simulink library "ConverterPlantLibrary"  (R2026a)
settings: Solver=VariableStepAuto
libraries: nesl_utility x213, fl_lib x211, ee_lib x205
(part 16 of 22)

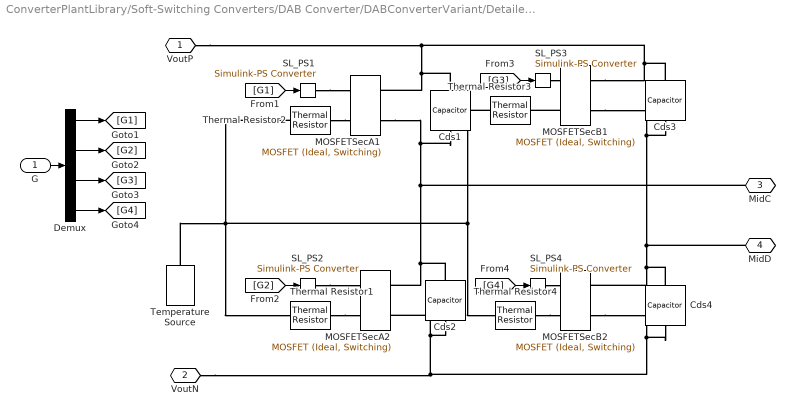
== system ConverterPlantLibrary/Soft-Switching Converters/DAB Converter/DABConverterVariant/DetailedModel/SecondaryBridge/SwitchingMOSFETwithThermal ==
  G : Inport
  Cds{1..4} (4 alike) : ee_lib/Passive/Capacitor  cap_option=ee.enum.passive.capacitor.capOption.const  c=CossSec_SI F  Cvec=[1e-05, 1e-06] F  Vvec=[0, 10] V  CV_table_symmetry=ee.enum.passive.capacitor.tableSymmetry.yes  f_vec=[1, 10] kHz  DFext_vec=[.8, 1.2]  enable_C_tol=ee.enum.toleranceApplication.none  averaging_period=0 s  C_tol=5  tol_distribution=ee.enum.toleranceDistribution.uniform  nSigma=4  r=0.001 Ohm  g=1e-5 1/Ohm  enable_operating_limits=ee.enum.enable.no  operating_limit_action=ee.enum.passive.reportOpLim.warn  max_working_voltage_range=[-25, 25] V  power_rating=1 W  maxTemperature=85 degC  thermalEnable=false  thermalMass=1 J/K  i_specify=off  i_priority=None  i=0 A  i_nominal_specify=off  i_nominal_value=1  i_nominal_unit=A  v_specify=off  v_priority=None  v=0 V  v_nominal_specify=off  v_nominal_value=1  v_nominal_unit=V  vc_specify=on  vc_priority=None  vc=0 V  vc_nominal_specify=off  vc_nominal_value=1  vc_nominal_unit=V  T_specify=off  T_priority=None  T=298.15 K  T_nominal_specify=off  T_nominal_value=1  T_nominal_unit=K
  Demux : Demux
  MOSFETSecA1 : ee_lib/Semiconductors & Converters/MOSFET (Ideal, Switching)  PartSpecification="{\"CollectionId\":\"MW.SimscapeElectrical\",\"CollectionVersion\":\"1.0.0\",\"DatasetId\":\"Wolfspeed|E4M0045075K1|\",\"DisplayName\":\"Wolfspeed:E4M0045075K1\"}"  port_option=ee.enum.controlport.ps  Rds=0.045 % Datasheet derived Ohm  Goff=1e-05 S  Vth=2.6 % Wolfspeed XML derived V  diode_param=ee.enum.converters.protectiondiode.nodynamics  diode_Vf=2.21 % Datasheet derived V  diode_Ron=0.02 % Wolfspeed XML derived Ohm  diode_Goff=1e-05 % Library default S  diode_C=50e-9 % Parameter not set F  diode_iRM=-235 % Parameter not set A  diode_iF=300 % Parameter not set A  diode_idot=-50 % Parameter not set A/us  diode_trr_param=ee.enum.converters.diodeReverseParam.trr_factor  diode_trr_factor=3 % Parameter not set  diode_trr=15 % Parameter not set us  diode_Qrr=1500 % Parameter not set s*uA  ids_specify=off  ids_priority=None  ids=0 A  ids_nominal_specify=off  ids_nominal_value=1  ids_nominal_unit=A  vds_specify=off  vds_priority=None  vds=0 V  vds_nominal_specify=off  vds_nominal_value=1  vds_nominal_unit=V  vgs_specify=off  vgs_priority=None  vgs=0 V  vgs_nominal_specify=off  vgs_nominal_value=1  vgs_nominal_unit=V  thermal_loss_option=ee.enum.converters.thermalLossOption.tabulated2d  Von_data=[-4.5606 -3.8186 -3.2298 -2.6407 -2.0162 -1.3202 -0.71619 -0.4914 -0.25251 -0.10121 -0.049071 0 0.046955 0.096318 0.24814 0.51166 0.78533 1.638 2.8067 4.0083;-6.1438 -4.6059 -3.5721 -2.779 -2.0216 -1.2551 -0.64969 -0.43829 -0.22166 -0.088463 -0.0434 0 0.04287 0.088364 0.22316 0.45399 0.69097 1.4423 2.5474 3.8258;-8.4687 -7.7777 -6.5652 -4.9559 -3.3669 -1.9919 -1.0021 -0.67224 -0.33819 -0.13631 -0.067471 0 0.066975 0.13508 0.34144 0.68685 1.0406 2.1699 3.9874 6.6428;-9.3156 -8.5555 -7.2218 -5.4514 -3.7036 -2.1911 -1.1023 -0.73946 -0.37201 -0.14994 -0.074218 0 0.073673 0.14859 0.37559 0.75553 1.1447 2.3869 4.3861 7.3071] % Wolfspeed XML derived V  Tj=[-55 25 175 900] % Wolfspeed XML derived degC  Iout_data=[-130 -110 -90 -70 -50 -30 -15 -10 -5 -2 -1 0 1 2 5 10 15 30 50 70] % Wolfspeed XML derived A  tabulateWithVds=false  Eon_data=[0 7.0888e-05 7.7152e-05 8.1716e-05 8.4697e-05 8.7728e-05 9.0888e-05 9.4243e-05 9.744e-05;0 7.7446e-05 8.2187e-05 8.4859e-05 8.6481e-05 8.8862e-05 9.0056e-05 9.2324e-05 9.4668e-05;0 7.794e-05 8.1085e-05 8.3317e-05 8.3898e-05 8.5847e-05 8.7874e-05 9.064e-05 9.3256e-05;0 7.7083e-05 7.9013e-05 8.0167e-05 8.1936e-05 8.4209e-05 8.8203e-05 9.1018e-05 9.9494e-05;0 8.4792e-05 8.6915e-05 8.8184e-05 9.013e-05 9.263e-05 9.7023e-05 0.00010012 0.00010944] % Wolfspeed XML derived J  Eoff_data=[0 2.4146e-05 1.5297e-05 1.3888e-05 1.7201e-05 2.1289e-05 2.6159e-05 3.3682e-05 4.1813e-05;0 2.543e-05 1.8251e-05 1.4144e-05 1.9418e-05 2.3393e-05 2.9608e-05 3.7025e-05 4.5856e-05;0 2.3401e-05 1.8149e-05 1.3882e-05 1.8943e-05 2.3112e-05 2.887e-05 3.79e-05 4.7249e-05;0 2.4371e-05 1.7115e-05 1.4404e-05 1.9523e-05 2.3993e-05 3.0691e-05 3.9068e-05 4.987e-05;0 2.6808e-05 1.8827e-05 1.5845e-05 2.1475e-05 2.6393e-05 3.376e-05 4.2974e-05 5.4857e-05] % Wolfspeed XML derived J  Eon_data_3D=reshape([0;0;0;0;0;0;0;0;0;0;0;0;0;0;0;0;0;0;0;0;0;0;0;0;0;0;0;0;0;0;0;0;0;0;0;0;0;0;0;0;0;0;0;0;0;0;0;0;0;0;0;0;0;0;0;0;0;0;0;0;0;0;0;0;0;0;0;0;0;0;0;0;0;0;0;0;0;0;0;0;0;0;0;0;0;0;0;0;0;0;0;0;0;0;0;7.0888e-05;7.7446e-05;7.794e-05;7.7083e-05;8.4792e-05;7.7152e-05;8.2187e-05;8.1085e-05;7.9013e-05;8.6915e-05;8.1716e-05;8.4859e-05;8.3317e-05;8.0167e-05;8.8184e-05;8.4697e-05;8.6481e-05;8.3898e-05;8.1936e-05;9.013e-05;8.7728e-05;8.8862e-05;8.5847e-05;8.4209e-05;9.263e-05;9.0888e-05;9.0056e-05;8.7874e-05;8.8203e-05;9.7023e-05;9.4243e-05;9.2324e-05;9.064e-05;9.1018e-05;0.00010012;9.744e-05;9.4668e-05;9.3256e-05;9.9494e-05;0.00010944],[5 9 3]) % Wolfspeed XML derived J  Eoff_data_3D=reshape([0;0;0;0;0;0;0;0;0;0;0;0;0;0;0;0;0;0;0;0;0;0;0;0;0;0;0;0;0;0;0;0;0;0;0;0;0;0;0;0;0;0;0;0;0;0;0;0;0;0;0;0;0;0;0;0;0;0;0;0;0;0;0;0;0;0;0;0;0;0;0;0;0;0;0;0;0;0;0;0;0;0;0;0;0;0;0;0;0;0;0;0;0;0;0;2.4146e-05;2.543e-05;2.3401e-05;2.4371e-05;2.6808e-05;1.5297e-05;1.8251e-05;1.8149e-05;1.7115e-05;1.8827e-05;1.3888e-05;1.4144e-05;1.3882e-05;1.4404e-05;1.5845e-05;1.7201e-05;1.9418e-05;1.8943e-05;1.9523e-05;2.1475e-05;2.1289e-05;2.3393e-05;2.3112e-05;2.3993e-05;2.6393e-05;2.6159e-05;2.9608e-05;2.887e-05;3.0691e-05;3.376e-05;3.3682e-05;3.7025e-05;3.79e-05;3.9068e-05;4.2974e-05;4.1813e-05;4.5856e-05;4.7249e-05;4.987e-05;5.4857e-05],[5 9 3]) % Wolfspeed XML derived J  Tj_loss=[25 75 125 175 900] % Wolfspeed XML derived degC  Iout_data_loss=[0 4.78844 9.555 13.3613 17.6794 21.5425 25.5456 29.2381 32.9963] % Wolfspeed XML derived A  Vds_loss=[-100 0 500] % Wolfspeed XML derived V  Eon_scalar=22.86e-3 % Parameter not set J  Eoff_scalar=17.14e-3 % Parameter not set J  Voff=300 % Parameter not set V  Iout_scalar=600 % Parameter not set A  useCurrentFromPreviousCycle=false % Parameter not set  useVoltageFromPreviousCycle=false % Parameter not set  diodeModelType=ee.enum.converters.diodeModelType.tabulated  diodeTableType=ee.enum.diode.tableType.VfMat  diode_ReverseIVType=ee.enum.diode.diodeReverseIV.constant  diode_IfMat=[.07, .12, .19, 1.75, 4.24, 7.32, 11.2; .16, .3, .72, 2.14, 4.02, 6.35, 9.12] % Parameter not set A  diode_VfMat=[0 3.93919 4.34166 5.03764 5.72176 6.19029 7.12243 7.9435 8.58508 9.13853 9.62104 10.0233;0 3.40354 3.71573 4.29235 4.91641 5.38167 6.38957 7.34226 8.07348 8.65657 9.13334 9.54153;0 2.99679 3.29251 3.84591 4.43945 4.88555 5.86847 6.80976 7.53945 8.14153 8.65715 9.11245;0 2.39743 2.63401 3.07672 3.55156 3.90844 4.69478 5.44781 6.03156 6.51323 6.92572 7.28996] % Wolfspeed XML derived V  diode_TjVec=[-55 25 175 900] % Wolfspeed XML derived degC  diode_VfVec=[.5, .7, .9, 1.3, 1.7, 2.1, 2.5] % Parameter not set V  diode_IfVec=[0 1 2 5 10 15 30 50 70 90 110 130] % Wolfspeed XML derived A  diode_IrMat=[1e-06, 2e-06, 5e-06, 1e-05, 2.5e-05, 5e-05, .0001; 2e-06, 5e-06, 1e-05, 4e-05, 8e-05, .0002, .0005] % Parameter not set A  diode_VrMat=[10, 100, 200, 250, 300, 325, 350; 10, 70, 160, 220, 270, 300, 320] % Parameter not set V  diode_VrVec=[10, 20, 40, 50, 70, 80, 100] % Parameter not set V  diode_IrVec=[1e-06, 2e-06, 5e-06, 1e-05, 2e-05, 5e-05, .0001] % Parameter not set A  diode_Vr=-600 % Parameter not set V  diode_Ls=150 % Parameter not set nH  diode_Erec=0.03 % Parameter not set J  diode_rec_loss_model=ee.enum.diode.reverseRecoveryModel.fixed  diode_ErecVal=0 % Parameter not set J  diode_scaleWithIandV=false  diode_ErecMat=[0 0;0 0] % Wolfspeed XML derived J  diodeErecMat3D=zeros(2, 3, 2) J  diode_TjrecVec=[25 35] % Wolfspeed XML derived degC  diode_IfrecVec=[0 10] % Wolfspeed XML derived A  diodeVrecVec=[0, 100] V  diode_IrecVal=10 % Parameter not set A  diode_VrecVal=10 % Wolfspeed XML derived V  diode_tFilter=1 / 1000 / 100 % Parameter not set s  separateThermalPortForDiode=false  thermal_network_parameterization=ee.enum.thermalNetworkTopology.external  Rth=[.03, .2] % Parameter not set K/W  Rth_Cauer=[0.089671 0.30799 0.22252 0.20902] % Wolfspeed XML derived K/W  Rth_Foster=[.08, .14, .22, .16] % Parameter not set K/W  thermal_mass_parameterization=ee.enum.thermalNetwork.thermalmass  thermal_mass=[3, 25] % Parameter not set J/K  thermal_mass_Cauer=[0.00092793 0.0041354 0.020593 0.15749] % Wolfspeed XML derived J/K  thermal_mass_Foster=[.001, .005, .05, .5] % Parameter not set J/K  thermal_time_constant=[.1, 5] % Parameter not set s  thermal_time_constant_Cauer=[.1, 1, 5] % Parameter not set s  thermal_time_constant_Foster=[7e-05, .0007, .01, .08] % Parameter not set s  thermal_mass_initial_temperatures=[25, 25] % Parameter not set degC  thermal_mass_initial_temperatures_Cauer=[25 25 25 25] % Wolfspeed XML derived degC  junction_thermal_mass=0.1 % Parameter not set J/K  Tvec_initial_Foster=[25, 25, 25, 25] % Parameter not set degC  RthDiode=[.03, .2] % Parameter not set K/W  RthCauerDiode=[0.089671 0.30799 0.22252 0.20902] % Wolfspeed XML derived K/W  RthFosterDiode=[.03, .2] % Parameter not set K/W  thermalMassDiode=[3, 25] % Parameter not set J/K  thermalMassCauerDiode=[0.00092793 0.0041354 0.020593 0.15749] % Wolfspeed XML derived J/K  thermalMassFosterDiode=[33, 50] % Parameter not set J/K  thermalTauDiode=[.1, 5] % Parameter not set s  thermalTauCauerDiode=[.1, 1, 5] % Parameter not set s  thermalTauFosterDiode=[1, 10] % Parameter not set s  thermalMassInitTempDiode=[25, 25] % Parameter not set degC  thermalMassInitTempCauerDiode=[25 25 25 25] % Wolfspeed XML derived degC  junctionthermalMassDiode=0.1 % Parameter not set J/K  TVecInitialFosterDiode=[25, 25, 25, 25] % Parameter not set degC  no_thermal_network=0 % Parameter not set  mosfet_junction_temperature_specify=on  mosfet_junction_temperature_priority=High  mosfet_junction_temperature=simTempSec_K K  mosfet_junction_temperature_nominal_specify=off  mosfet_junction_temperature_nominal_value=1  mosfet_junction_temperature_nominal_unit=degC  diode_junction_temperature_specify=off  diode_junction_temperature_priority=None  diode_junction_temperature=simTempSec_K K  diode_junction_temperature_nominal_specify=off  diode_junction_temperature_nominal_value=1  diode_junction_temperature_nominal_unit=degC  Qj_specify=off  Qj_priority=None  Qj=0 W  Qj_nominal_specify=off  Qj_nominal_value=1  Qj_nominal_unit=W  accumulatedSwitchingLosses_specify=off  accumulatedSwitchingLosses_priority=None  accumulatedSwitchingLosses=0 J
      settings: AttributesFormatString=Wolfspeed:E4M0045075K1
  MOSFETSecA2 : ee_lib/Semiconductors & Converters/MOSFET (Ideal, Switching)  port_option=ee.enum.controlport.ps  Rds=0.045 % Datasheet derived Ohm  Goff=1e-05 S  Vth=2.6 % Wolfspeed XML derived V  diode_param=ee.enum.converters.protectiondiode.nodynamics  diode_Vf=2.21 % Datasheet derived V  diode_Ron=0.02 % Wolfspeed XML derived Ohm  diode_Goff=1e-05 % Library default S  diode_C=50e-9 % Parameter not set F  diode_iRM=-235 % Parameter not set A  diode_iF=300 % Parameter not set A  diode_idot=-50 % Parameter not set A/us  diode_trr_param=ee.enum.converters.diodeReverseParam.trr_factor  diode_trr_factor=3 % Parameter not set  diode_trr=15 % Parameter not set us  diode_Qrr=1500 % Parameter not set s*uA  ids_specify=off  ids_priority=None  ids=0 A  ids_nominal_specify=off  ids_nominal_value=1  ids_nominal_unit=A  vds_specify=off  vds_priority=None  vds=0 V  vds_nominal_specify=off  vds_nominal_value=1  vds_nominal_unit=V  vgs_specify=off  vgs_priority=None  vgs=0 V  vgs_nominal_specify=off  vgs_nominal_value=1  vgs_nominal_unit=V  thermal_loss_option=ee.enum.converters.thermalLossOption.tabulated2d  Von_data=[-4.5606 -3.8186 -3.2298 -2.6407 -2.0162 -1.3202 -0.71619 -0.4914 -0.25251 -0.10121 -0.049071 0 0.046955 0.096318 0.24814 0.51166 0.78533 1.638 2.8067 4.0083;-6.1438 -4.6059 -3.5721 -2.779 -2.0216 -1.2551 -0.64969 -0.43829 -0.22166 -0.088463 -0.0434 0 0.04287 0.088364 0.22316 0.45399 0.69097 1.4423 2.5474 3.8258;-8.4687 -7.7777 -6.5652 -4.9559 -3.3669 -1.9919 -1.0021 -0.67224 -0.33819 -0.13631 -0.067471 0 0.066975 0.13508 0.34144 0.68685 1.0406 2.1699 3.9874 6.6428;-9.3156 -8.5555 -7.2218 -5.4514 -3.7036 -2.1911 -1.1023 -0.73946 -0.37201 -0.14994 -0.074218 0 0.073673 0.14859 0.37559 0.75553 1.1447 2.3869 4.3861 7.3071] % Wolfspeed XML derived V  Tj=[-55 25 175 900] % Wolfspeed XML derived degC  Iout_data=[-130 -110 -90 -70 -50 -30 -15 -10 -5 -2 -1 0 1 2 5 10 15 30 50 70] % Wolfspeed XML derived A  tabulateWithVds=false  Eon_data=[0 7.0888e-05 7.7152e-05 8.1716e-05 8.4697e-05 8.7728e-05 9.0888e-05 9.4243e-05 9.744e-05;0 7.7446e-05 8.2187e-05 8.4859e-05 8.6481e-05 8.8862e-05 9.0056e-05 9.2324e-05 9.4668e-05;0 7.794e-05 8.1085e-05 8.3317e-05 8.3898e-05 8.5847e-05 8.7874e-05 9.064e-05 9.3256e-05;0 7.7083e-05 7.9013e-05 8.0167e-05 8.1936e-05 8.4209e-05 8.8203e-05 9.1018e-05 9.9494e-05;0 8.4792e-05 8.6915e-05 8.8184e-05 9.013e-05 9.263e-05 9.7023e-05 0.00010012 0.00010944] % Wolfspeed XML derived J  Eoff_data=[0 2.4146e-05 1.5297e-05 1.3888e-05 1.7201e-05 2.1289e-05 2.6159e-05 3.3682e-05 4.1813e-05;0 2.543e-05 1.8251e-05 1.4144e-05 1.9418e-05 2.3393e-05 2.9608e-05 3.7025e-05 4.5856e-05;0 2.3401e-05 1.8149e-05 1.3882e-05 1.8943e-05 2.3112e-05 2.887e-05 3.79e-05 4.7249e-05;0 2.4371e-05 1.7115e-05 1.4404e-05 1.9523e-05 2.3993e-05 3.0691e-05 3.9068e-05 4.987e-05;0 2.6808e-05 1.8827e-05 1.5845e-05 2.1475e-05 2.6393e-05 3.376e-05 4.2974e-05 5.4857e-05] % Wolfspeed XML derived J  Eon_data_3D=reshape([0;0;0;0;0;0;0;0;0;0;0;0;0;0;0;0;0;0;0;0;0;0;0;0;0;0;0;0;0;0;0;0;0;0;0;0;0;0;0;0;0;0;0;0;0;0;0;0;0;0;0;0;0;0;0;0;0;0;0;0;0;0;0;0;0;0;0;0;0;0;0;0;0;0;0;0;0;0;0;0;0;0;0;0;0;0;0;0;0;0;0;0;0;0;0;7.0888e-05;7.7446e-05;7.794e-05;7.7083e-05;8.4792e-05;7.7152e-05;8.2187e-05;8.1085e-05;7.9013e-05;8.6915e-05;8.1716e-05;8.4859e-05;8.3317e-05;8.0167e-05;8.8184e-05;8.4697e-05;8.6481e-05;8.3898e-05;8.1936e-05;9.013e-05;8.7728e-05;8.8862e-05;8.5847e-05;8.4209e-05;9.263e-05;9.0888e-05;9.0056e-05;8.7874e-05;8.8203e-05;9.7023e-05;9.4243e-05;9.2324e-05;9.064e-05;9.1018e-05;0.00010012;9.744e-05;9.4668e-05;9.3256e-05;9.9494e-05;0.00010944],[5 9 3]) % Wolfspeed XML derived J  Eoff_data_3D=reshape([0;0;0;0;0;0;0;0;0;0;0;0;0;0;0;0;0;0;0;0;0;0;0;0;0;0;0;0;0;0;0;0;0;0;0;0;0;0;0;0;0;0;0;0;0;0;0;0;0;0;0;0;0;0;0;0;0;0;0;0;0;0;0;0;0;0;0;0;0;0;0;0;0;0;0;0;0;0;0;0;0;0;0;0;0;0;0;0;0;0;0;0;0;0;0;2.4146e-05;2.543e-05;2.3401e-05;2.4371e-05;2.6808e-05;1.5297e-05;1.8251e-05;1.8149e-05;1.7115e-05;1.8827e-05;1.3888e-05;1.4144e-05;1.3882e-05;1.4404e-05;1.5845e-05;1.7201e-05;1.9418e-05;1.8943e-05;1.9523e-05;2.1475e-05;2.1289e-05;2.3393e-05;2.3112e-05;2.3993e-05;2.6393e-05;2.6159e-05;2.9608e-05;2.887e-05;3.0691e-05;3.376e-05;3.3682e-05;3.7025e-05;3.79e-05;3.9068e-05;4.2974e-05;4.1813e-05;4.5856e-05;4.7249e-05;4.987e-05;5.4857e-05],[5 9 3]) % Wolfspeed XML derived J  Tj_loss=[25 75 125 175 900] % Wolfspeed XML derived degC  Iout_data_loss=[0 4.78844 9.555 13.3613 17.6794 21.5425 25.5456 29.2381 32.9963] % Wolfspeed XML derived A  Vds_loss=[-100 0 500] % Wolfspeed XML derived V  Eon_scalar=22.86e-3 % Parameter not set J  Eoff_scalar=17.14e-3 % Parameter not set J  Voff=300 % Parameter not set V  Iout_scalar=600 % Parameter not set A  useCurrentFromPreviousCycle=false % Parameter not set  useVoltageFromPreviousCycle=false % Parameter not set  diodeModelType=ee.enum.converters.diodeModelType.tabulated  diodeTableType=ee.enum.diode.tableType.VfMat  diode_ReverseIVType=ee.enum.diode.diodeReverseIV.constant  diode_IfMat=[.07, .12, .19, 1.75, 4.24, 7.32, 11.2; .16, .3, .72, 2.14, 4.02, 6.35, 9.12] % Parameter not set A  diode_VfMat=[0 3.93919 4.34166 5.03764 5.72176 6.19029 7.12243 7.9435 8.58508 9.13853 9.62104 10.0233;0 3.40354 3.71573 4.29235 4.91641 5.38167 6.38957 7.34226 8.07348 8.65657 9.13334 9.54153;0 2.99679 3.29251 3.84591 4.43945 4.88555 5.86847 6.80976 7.53945 8.14153 8.65715 9.11245;0 2.39743 2.63401 3.07672 3.55156 3.90844 4.69478 5.44781 6.03156 6.51323 6.92572 7.28996] % Wolfspeed XML derived V  diode_TjVec=[-55 25 175 900] % Wolfspeed XML derived degC  diode_VfVec=[.5, .7, .9, 1.3, 1.7, 2.1, 2.5] % Parameter not set V  diode_IfVec=[0 1 2 5 10 15 30 50 70 90 110 130] % Wolfspeed XML derived A  diode_IrMat=[1e-06, 2e-06, 5e-06, 1e-05, 2.5e-05, 5e-05, .0001; 2e-06, 5e-06, 1e-05, 4e-05, 8e-05, .0002, .0005] % Parameter not set A  diode_VrMat=[10, 100, 200, 250, 300, 325, 350; 10, 70, 160, 220, 270, 300, 320] % Parameter not set V  diode_VrVec=[10, 20, 40, 50, 70, 80, 100] % Parameter not set V  diode_IrVec=[1e-06, 2e-06, 5e-06, 1e-05, 2e-05, 5e-05, .0001] % Parameter not set A  diode_Vr=-600 % Parameter not set V  diode_Ls=150 % Parameter not set nH  diode_Erec=0.03 % Parameter not set J  diode_rec_loss_model=ee.enum.diode.reverseRecoveryModel.fixed  diode_ErecVal=0 % Parameter not set J  diode_scaleWithIandV=false  diode_ErecMat=[0 0;0 0] % Wolfspeed XML derived J  diodeErecMat3D=zeros(2, 3, 2) J  diode_TjrecVec=[25 35] % Wolfspeed XML derived degC  diode_IfrecVec=[0 10] % Wolfspeed XML derived A  diodeVrecVec=[0, 100] V  diode_IrecVal=10 % Parameter not set A  diode_VrecVal=10 % Wolfspeed XML derived V  diode_tFilter=1 / 1000 / 100 % Parameter not set s  separateThermalPortForDiode=false  thermal_network_parameterization=ee.enum.thermalNetworkTopology.external  Rth=[.03, .2] % Parameter not set K/W  Rth_Cauer=[0.089671 0.30799 0.22252 0.20902] % Wolfspeed XML derived K/W  Rth_Foster=[.08, .14, .22, .16] % Parameter not set K/W  thermal_mass_parameterization=ee.enum.thermalNetwork.thermalmass  thermal_mass=[3, 25] % Parameter not set J/K  thermal_mass_Cauer=[0.00092793 0.0041354 0.020593 0.15749] % Wolfspeed XML derived J/K  thermal_mass_Foster=[.001, .005, .05, .5] % Parameter not set J/K  thermal_time_constant=[.1, 5] % Parameter not set s  thermal_time_constant_Cauer=[.1, 1, 5] % Parameter not set s  thermal_time_constant_Foster=[7e-05, .0007, .01, .08] % Parameter not set s  thermal_mass_initial_temperatures=[25, 25] % Parameter not set degC  thermal_mass_initial_temperatures_Cauer=[25 25 25 25] % Wolfspeed XML derived degC  junction_thermal_mass=0.1 % Parameter not set J/K  Tvec_initial_Foster=[25, 25, 25, 25] % Parameter not set degC  RthDiode=[.03, .2] % Parameter not set K/W  RthCauerDiode=[0.089671 0.30799 0.22252 0.20902] % Wolfspeed XML derived K/W  RthFosterDiode=[.03, .2] % Parameter not set K/W  thermalMassDiode=[3, 25] % Parameter not set J/K  thermalMassCauerDiode=[0.00092793 0.0041354 0.020593 0.15749] % Wolfspeed XML derived J/K  thermalMassFosterDiode=[33, 50] % Parameter not set J/K  thermalTauDiode=[.1, 5] % Parameter not set s  thermalTauCauerDiode=[.1, 1, 5] % Parameter not set s  thermalTauFosterDiode=[1, 10] % Parameter not set s  thermalMassInitTempDiode=[25, 25] % Parameter not set degC  thermalMassInitTempCauerDiode=[25 25 25 25] % Wolfspeed XML derived degC  junctionthermalMassDiode=0.1 % Parameter not set J/K  TVecInitialFosterDiode=[25, 25, 25, 25] % Parameter not set degC  no_thermal_network=0 % Parameter not set  mosfet_junction_temperature_specify=on  mosfet_junction_temperature_priority=High  mosfet_junction_temperature=simTempSec_K K  mosfet_junction_temperature_nominal_specify=off  mosfet_junction_temperature_nominal_value=1  mosfet_junction_temperature_nominal_unit=degC  diode_junction_temperature_specify=off  diode_junction_temperature_priority=None  diode_junction_temperature=simTempSec_K K  diode_junction_temperature_nominal_specify=off  diode_junction_temperature_nominal_value=1  diode_junction_temperature_nominal_unit=degC  Qj_specify=off  Qj_priority=None  Qj=0 W  Qj_nominal_specify=off  Qj_nominal_value=1  Qj_nominal_unit=W  accumulatedSwitchingLosses_specify=off  accumulatedSwitchingLosses_priority=None  accumulatedSwitchingLosses=0 J
  MOSFETSecB1 : ee_lib/Semiconductors & Converters/MOSFET (Ideal, Switching)  port_option=ee.enum.controlport.ps  Rds=0.045 % Datasheet derived Ohm  Goff=1e-05 S  Vth=2.6 % Wolfspeed XML derived V  diode_param=ee.enum.converters.protectiondiode.nodynamics  diode_Vf=2.21 % Datasheet derived V  diode_Ron=0.02 % Wolfspeed XML derived Ohm  diode_Goff=1e-05 % Library default S  diode_C=50e-9 % Parameter not set F  diode_iRM=-235 % Parameter not set A  diode_iF=300 % Parameter not set A  diode_idot=-50 % Parameter not set A/us  diode_trr_param=ee.enum.converters.diodeReverseParam.trr_factor  diode_trr_factor=3 % Parameter not set  diode_trr=15 % Parameter not set us  diode_Qrr=1500 % Parameter not set s*uA  ids_specify=off  ids_priority=None  ids=0 A  ids_nominal_specify=off  ids_nominal_value=1  ids_nominal_unit=A  vds_specify=off  vds_priority=None  vds=0 V  vds_nominal_specify=off  vds_nominal_value=1  vds_nominal_unit=V  vgs_specify=off  vgs_priority=None  vgs=0 V  vgs_nominal_specify=off  vgs_nominal_value=1  vgs_nominal_unit=V  thermal_loss_option=ee.enum.converters.thermalLossOption.tabulated2d  Von_data=[-4.5606 -3.8186 -3.2298 -2.6407 -2.0162 -1.3202 -0.71619 -0.4914 -0.25251 -0.10121 -0.049071 0 0.046955 0.096318 0.24814 0.51166 0.78533 1.638 2.8067 4.0083;-6.1438 -4.6059 -3.5721 -2.779 -2.0216 -1.2551 -0.64969 -0.43829 -0.22166 -0.088463 -0.0434 0 0.04287 0.088364 0.22316 0.45399 0.69097 1.4423 2.5474 3.8258;-8.4687 -7.7777 -6.5652 -4.9559 -3.3669 -1.9919 -1.0021 -0.67224 -0.33819 -0.13631 -0.067471 0 0.066975 0.13508 0.34144 0.68685 1.0406 2.1699 3.9874 6.6428;-9.3156 -8.5555 -7.2218 -5.4514 -3.7036 -2.1911 -1.1023 -0.73946 -0.37201 -0.14994 -0.074218 0 0.073673 0.14859 0.37559 0.75553 1.1447 2.3869 4.3861 7.3071] % Wolfspeed XML derived V  Tj=[-55 25 175 900] % Wolfspeed XML derived degC  Iout_data=[-130 -110 -90 -70 -50 -30 -15 -10 -5 -2 -1 0 1 2 5 10 15 30 50 70] % Wolfspeed XML derived A  tabulateWithVds=false  Eon_data=[0 7.0888e-05 7.7152e-05 8.1716e-05 8.4697e-05 8.7728e-05 9.0888e-05 9.4243e-05 9.744e-05;0 7.7446e-05 8.2187e-05 8.4859e-05 8.6481e-05 8.8862e-05 9.0056e-05 9.2324e-05 9.4668e-05;0 7.794e-05 8.1085e-05 8.3317e-05 8.3898e-05 8.5847e-05 8.7874e-05 9.064e-05 9.3256e-05;0 7.7083e-05 7.9013e-05 8.0167e-05 8.1936e-05 8.4209e-05 8.8203e-05 9.1018e-05 9.9494e-05;0 8.4792e-05 8.6915e-05 8.8184e-05 9.013e-05 9.263e-05 9.7023e-05 0.00010012 0.00010944] % Wolfspeed XML derived J  Eoff_data=[0 2.4146e-05 1.5297e-05 1.3888e-05 1.7201e-05 2.1289e-05 2.6159e-05 3.3682e-05 4.1813e-05;0 2.543e-05 1.8251e-05 1.4144e-05 1.9418e-05 2.3393e-05 2.9608e-05 3.7025e-05 4.5856e-05;0 2.3401e-05 1.8149e-05 1.3882e-05 1.8943e-05 2.3112e-05 2.887e-05 3.79e-05 4.7249e-05;0 2.4371e-05 1.7115e-05 1.4404e-05 1.9523e-05 2.3993e-05 3.0691e-05 3.9068e-05 4.987e-05;0 2.6808e-05 1.8827e-05 1.5845e-05 2.1475e-05 2.6393e-05 3.376e-05 4.2974e-05 5.4857e-05] % Wolfspeed XML derived J  Eon_data_3D=reshape([0;0;0;0;0;0;0;0;0;0;0;0;0;0;0;0;0;0;0;0;0;0;0;0;0;0;0;0;0;0;0;0;0;0;0;0;0;0;0;0;0;0;0;0;0;0;0;0;0;0;0;0;0;0;0;0;0;0;0;0;0;0;0;0;0;0;0;0;0;0;0;0;0;0;0;0;0;0;0;0;0;0;0;0;0;0;0;0;0;0;0;0;0;0;0;7.0888e-05;7.7446e-05;7.794e-05;7.7083e-05;8.4792e-05;7.7152e-05;8.2187e-05;8.1085e-05;7.9013e-05;8.6915e-05;8.1716e-05;8.4859e-05;8.3317e-05;8.0167e-05;8.8184e-05;8.4697e-05;8.6481e-05;8.3898e-05;8.1936e-05;9.013e-05;8.7728e-05;8.8862e-05;8.5847e-05;8.4209e-05;9.263e-05;9.0888e-05;9.0056e-05;8.7874e-05;8.8203e-05;9.7023e-05;9.4243e-05;9.2324e-05;9.064e-05;9.1018e-05;0.00010012;9.744e-05;9.4668e-05;9.3256e-05;9.9494e-05;0.00010944],[5 9 3]) % Wolfspeed XML derived J  Eoff_data_3D=reshape([0;0;0;0;0;0;0;0;0;0;0;0;0;0;0;0;0;0;0;0;0;0;0;0;0;0;0;0;0;0;0;0;0;0;0;0;0;0;0;0;0;0;0;0;0;0;0;0;0;0;0;0;0;0;0;0;0;0;0;0;0;0;0;0;0;0;0;0;0;0;0;0;0;0;0;0;0;0;0;0;0;0;0;0;0;0;0;0;0;0;0;0;0;0;0;2.4146e-05;2.543e-05;2.3401e-05;2.4371e-05;2.6808e-05;1.5297e-05;1.8251e-05;1.8149e-05;1.7115e-05;1.8827e-05;1.3888e-05;1.4144e-05;1.3882e-05;1.4404e-05;1.5845e-05;1.7201e-05;1.9418e-05;1.8943e-05;1.9523e-05;2.1475e-05;2.1289e-05;2.3393e-05;2.3112e-05;2.3993e-05;2.6393e-05;2.6159e-05;2.9608e-05;2.887e-05;3.0691e-05;3.376e-05;3.3682e-05;3.7025e-05;3.79e-05;3.9068e-05;4.2974e-05;4.1813e-05;4.5856e-05;4.7249e-05;4.987e-05;5.4857e-05],[5 9 3]) % Wolfspeed XML derived J  Tj_loss=[25 75 125 175 900] % Wolfspeed XML derived degC  Iout_data_loss=[0 4.78844 9.555 13.3613 17.6794 21.5425 25.5456 29.2381 32.9963] % Wolfspeed XML derived A  Vds_loss=[-100 0 500] % Wolfspeed XML derived V  Eon_scalar=22.86e-3 % Parameter not set J  Eoff_scalar=17.14e-3 % Parameter not set J  Voff=300 % Parameter not set V  Iout_scalar=600 % Parameter not set A  useCurrentFromPreviousCycle=false % Parameter not set  useVoltageFromPreviousCycle=false % Parameter not set  diodeModelType=ee.enum.converters.diodeModelType.tabulated  diodeTableType=ee.enum.diode.tableType.VfMat  diode_ReverseIVType=ee.enum.diode.diodeReverseIV.constant  diode_IfMat=[.07, .12, .19, 1.75, 4.24, 7.32, 11.2; .16, .3, .72, 2.14, 4.02, 6.35, 9.12] % Parameter not set A  diode_VfMat=[0 3.93919 4.34166 5.03764 5.72176 6.19029 7.12243 7.9435 8.58508 9.13853 9.62104 10.0233;0 3.40354 3.71573 4.29235 4.91641 5.38167 6.38957 7.34226 8.07348 8.65657 9.13334 9.54153;0 2.99679 3.29251 3.84591 4.43945 4.88555 5.86847 6.80976 7.53945 8.14153 8.65715 9.11245;0 2.39743 2.63401 3.07672 3.55156 3.90844 4.69478 5.44781 6.03156 6.51323 6.92572 7.28996] % Wolfspeed XML derived V  diode_TjVec=[-55 25 175 900] % Wolfspeed XML derived degC  diode_VfVec=[.5, .7, .9, 1.3, 1.7, 2.1, 2.5] % Parameter not set V  diode_IfVec=[0 1 2 5 10 15 30 50 70 90 110 130] % Wolfspeed XML derived A  diode_IrMat=[1e-06, 2e-06, 5e-06, 1e-05, 2.5e-05, 5e-05, .0001; 2e-06, 5e-06, 1e-05, 4e-05, 8e-05, .0002, .0005] % Parameter not set A  diode_VrMat=[10, 100, 200, 250, 300, 325, 350; 10, 70, 160, 220, 270, 300, 320] % Parameter not set V  diode_VrVec=[10, 20, 40, 50, 70, 80, 100] % Parameter not set V  diode_IrVec=[1e-06, 2e-06, 5e-06, 1e-05, 2e-05, 5e-05, .0001] % Parameter not set A  diode_Vr=-600 % Parameter not set V  diode_Ls=150 % Parameter not set nH  diode_Erec=0.03 % Parameter not set J  diode_rec_loss_model=ee.enum.diode.reverseRecoveryModel.fixed  diode_ErecVal=0 % Parameter not set J  diode_scaleWithIandV=false  diode_ErecMat=[0 0;0 0] % Wolfspeed XML derived J  diodeErecMat3D=zeros(2, 3, 2) J  diode_TjrecVec=[25 35] % Wolfspeed XML derived degC  diode_IfrecVec=[0 10] % Wolfspeed XML derived A  diodeVrecVec=[0, 100] V  diode_IrecVal=10 % Parameter not set A  diode_VrecVal=10 % Wolfspeed XML derived V  diode_tFilter=1 / 1000 / 100 % Parameter not set s  separateThermalPortForDiode=false  thermal_network_parameterization=ee.enum.thermalNetworkTopology.external  Rth=[.03, .2] % Parameter not set K/W  Rth_Cauer=[0.089671 0.30799 0.22252 0.20902] % Wolfspeed XML derived K/W  Rth_Foster=[.08, .14, .22, .16] % Parameter not set K/W  thermal_mass_parameterization=ee.enum.thermalNetwork.thermalmass  thermal_mass=[3, 25] % Parameter not set J/K  thermal_mass_Cauer=[0.00092793 0.0041354 0.020593 0.15749] % Wolfspeed XML derived J/K  thermal_mass_Foster=[.001, .005, .05, .5] % Parameter not set J/K  thermal_time_constant=[.1, 5] % Parameter not set s  thermal_time_constant_Cauer=[.1, 1, 5] % Parameter not set s  thermal_time_constant_Foster=[7e-05, .0007, .01, .08] % Parameter not set s  thermal_mass_initial_temperatures=[25, 25] % Parameter not set degC  thermal_mass_initial_temperatures_Cauer=[25 25 25 25] % Wolfspeed XML derived degC  junction_thermal_mass=0.1 % Parameter not set J/K  Tvec_initial_Foster=[25, 25, 25, 25] % Parameter not set degC  RthDiode=[.03, .2] % Parameter not set K/W  RthCauerDiode=[0.089671 0.30799 0.22252 0.20902] % Wolfspeed XML derived K/W  RthFosterDiode=[.03, .2] % Parameter not set K/W  thermalMassDiode=[3, 25] % Parameter not set J/K  thermalMassCauerDiode=[0.00092793 0.0041354 0.020593 0.15749] % Wolfspeed XML derived J/K  thermalMassFosterDiode=[33, 50] % Parameter not set J/K  thermalTauDiode=[.1, 5] % Parameter not set s  thermalTauCauerDiode=[.1, 1, 5] % Parameter not set s  thermalTauFosterDiode=[1, 10] % Parameter not set s  thermalMassInitTempDiode=[25, 25] % Parameter not set degC  thermalMassInitTempCauerDiode=[25 25 25 25] % Wolfspeed XML derived degC  junctionthermalMassDiode=0.1 % Parameter not set J/K  TVecInitialFosterDiode=[25, 25, 25, 25] % Parameter not set degC  no_thermal_network=0 % Parameter not set  mosfet_junction_temperature_specify=on  mosfet_junction_temperature_priority=High  mosfet_junction_temperature=simTempSec_K K  mosfet_junction_temperature_nominal_specify=off  mosfet_junction_temperature_nominal_value=1  mosfet_junction_temperature_nominal_unit=degC  diode_junction_temperature_specify=off  diode_junction_temperature_priority=None  diode_junction_temperature=simTempSec_K K  diode_junction_temperature_nominal_specify=off  diode_junction_temperature_nominal_value=1  diode_junction_temperature_nominal_unit=degC  Qj_specify=off  Qj_priority=None  Qj=0 W  Qj_nominal_specify=off  Qj_nominal_value=1  Qj_nominal_unit=W  accumulatedSwitchingLosses_specify=off  accumulatedSwitchingLosses_priority=None  accumulatedSwitchingLosses=0 J
  MOSFETSecB2 : ee_lib/Semiconductors & Converters/MOSFET (Ideal, Switching)  port_option=ee.enum.controlport.ps  Rds=0.045 % Datasheet derived Ohm  Goff=1e-05 S  Vth=2.6 % Wolfspeed XML derived V  diode_param=ee.enum.converters.protectiondiode.nodynamics  diode_Vf=2.21 % Datasheet derived V  diode_Ron=0.02 % Wolfspeed XML derived Ohm  diode_Goff=1e-05 % Library default S  diode_C=50e-9 % Parameter not set F  diode_iRM=-235 % Parameter not set A  diode_iF=300 % Parameter not set A  diode_idot=-50 % Parameter not set A/us  diode_trr_param=ee.enum.converters.diodeReverseParam.trr_factor  diode_trr_factor=3 % Parameter not set  diode_trr=15 % Parameter not set us  diode_Qrr=1500 % Parameter not set s*uA  ids_specify=off  ids_priority=None  ids=0 A  ids_nominal_specify=off  ids_nominal_value=1  ids_nominal_unit=A  vds_specify=off  vds_priority=None  vds=0 V  vds_nominal_specify=off  vds_nominal_value=1  vds_nominal_unit=V  vgs_specify=off  vgs_priority=None  vgs=0 V  vgs_nominal_specify=off  vgs_nominal_value=1  vgs_nominal_unit=V  thermal_loss_option=ee.enum.converters.thermalLossOption.tabulated2d  Von_data=[-4.5606 -3.8186 -3.2298 -2.6407 -2.0162 -1.3202 -0.71619 -0.4914 -0.25251 -0.10121 -0.049071 0 0.046955 0.096318 0.24814 0.51166 0.78533 1.638 2.8067 4.0083;-6.1438 -4.6059 -3.5721 -2.779 -2.0216 -1.2551 -0.64969 -0.43829 -0.22166 -0.088463 -0.0434 0 0.04287 0.088364 0.22316 0.45399 0.69097 1.4423 2.5474 3.8258;-8.4687 -7.7777 -6.5652 -4.9559 -3.3669 -1.9919 -1.0021 -0.67224 -0.33819 -0.13631 -0.067471 0 0.066975 0.13508 0.34144 0.68685 1.0406 2.1699 3.9874 6.6428;-9.3156 -8.5555 -7.2218 -5.4514 -3.7036 -2.1911 -1.1023 -0.73946 -0.37201 -0.14994 -0.074218 0 0.073673 0.14859 0.37559 0.75553 1.1447 2.3869 4.3861 7.3071] % Wolfspeed XML derived V  Tj=[-55 25 175 900] % Wolfspeed XML derived degC  Iout_data=[-130 -110 -90 -70 -50 -30 -15 -10 -5 -2 -1 0 1 2 5 10 15 30 50 70] % Wolfspeed XML derived A  tabulateWithVds=false  Eon_data=[0 7.0888e-05 7.7152e-05 8.1716e-05 8.4697e-05 8.7728e-05 9.0888e-05 9.4243e-05 9.744e-05;0 7.7446e-05 8.2187e-05 8.4859e-05 8.6481e-05 8.8862e-05 9.0056e-05 9.2324e-05 9.4668e-05;0 7.794e-05 8.1085e-05 8.3317e-05 8.3898e-05 8.5847e-05 8.7874e-05 9.064e-05 9.3256e-05;0 7.7083e-05 7.9013e-05 8.0167e-05 8.1936e-05 8.4209e-05 8.8203e-05 9.1018e-05 9.9494e-05;0 8.4792e-05 8.6915e-05 8.8184e-05 9.013e-05 9.263e-05 9.7023e-05 0.00010012 0.00010944] % Wolfspeed XML derived J  Eoff_data=[0 2.4146e-05 1.5297e-05 1.3888e-05 1.7201e-05 2.1289e-05 2.6159e-05 3.3682e-05 4.1813e-05;0 2.543e-05 1.8251e-05 1.4144e-05 1.9418e-05 2.3393e-05 2.9608e-05 3.7025e-05 4.5856e-05;0 2.3401e-05 1.8149e-05 1.3882e-05 1.8943e-05 2.3112e-05 2.887e-05 3.79e-05 4.7249e-05;0 2.4371e-05 1.7115e-05 1.4404e-05 1.9523e-05 2.3993e-05 3.0691e-05 3.9068e-05 4.987e-05;0 2.6808e-05 1.8827e-05 1.5845e-05 2.1475e-05 2.6393e-05 3.376e-05 4.2974e-05 5.4857e-05] % Wolfspeed XML derived J  Eon_data_3D=reshape([0;0;0;0;0;0;0;0;0;0;0;0;0;0;0;0;0;0;0;0;0;0;0;0;0;0;0;0;0;0;0;0;0;0;0;0;0;0;0;0;0;0;0;0;0;0;0;0;0;0;0;0;0;0;0;0;0;0;0;0;0;0;0;0;0;0;0;0;0;0;0;0;0;0;0;0;0;0;0;0;0;0;0;0;0;0;0;0;0;0;0;0;0;0;0;7.0888e-05;7.7446e-05;7.794e-05;7.7083e-05;8.4792e-05;7.7152e-05;8.2187e-05;8.1085e-05;7.9013e-05;8.6915e-05;8.1716e-05;8.4859e-05;8.3317e-05;8.0167e-05;8.8184e-05;8.4697e-05;8.6481e-05;8.3898e-05;8.1936e-05;9.013e-05;8.7728e-05;8.8862e-05;8.5847e-05;8.4209e-05;9.263e-05;9.0888e-05;9.0056e-05;8.7874e-05;8.8203e-05;9.7023e-05;9.4243e-05;9.2324e-05;9.064e-05;9.1018e-05;0.00010012;9.744e-05;9.4668e-05;9.3256e-05;9.9494e-05;0.00010944],[5 9 3]) % Wolfspeed XML derived J  Eoff_data_3D=reshape([0;0;0;0;0;0;0;0;0;0;0;0;0;0;0;0;0;0;0;0;0;0;0;0;0;0;0;0;0;0;0;0;0;0;0;0;0;0;0;0;0;0;0;0;0;0;0;0;0;0;0;0;0;0;0;0;0;0;0;0;0;0;0;0;0;0;0;0;0;0;0;0;0;0;0;0;0;0;0;0;0;0;0;0;0;0;0;0;0;0;0;0;0;0;0;2.4146e-05;2.543e-05;2.3401e-05;2.4371e-05;2.6808e-05;1.5297e-05;1.8251e-05;1.8149e-05;1.7115e-05;1.8827e-05;1.3888e-05;1.4144e-05;1.3882e-05;1.4404e-05;1.5845e-05;1.7201e-05;1.9418e-05;1.8943e-05;1.9523e-05;2.1475e-05;2.1289e-05;2.3393e-05;2.3112e-05;2.3993e-05;2.6393e-05;2.6159e-05;2.9608e-05;2.887e-05;3.0691e-05;3.376e-05;3.3682e-05;3.7025e-05;3.79e-05;3.9068e-05;4.2974e-05;4.1813e-05;4.5856e-05;4.7249e-05;4.987e-05;5.4857e-05],[5 9 3]) % Wolfspeed XML derived J  Tj_loss=[25 75 125 175 900] % Wolfspeed XML derived degC  Iout_data_loss=[0 4.78844 9.555 13.3613 17.6794 21.5425 25.5456 29.2381 32.9963] % Wolfspeed XML derived A  Vds_loss=[-100 0 500] % Wolfspeed XML derived V  Eon_scalar=22.86e-3 % Parameter not set J  Eoff_scalar=17.14e-3 % Parameter not set J  Voff=300 % Parameter not set V  Iout_scalar=600 % Parameter not set A  useCurrentFromPreviousCycle=false % Parameter not set  useVoltageFromPreviousCycle=false % Parameter not set  diodeModelType=ee.enum.converters.diodeModelType.tabulated  diodeTableType=ee.enum.diode.tableType.VfMat  diode_ReverseIVType=ee.enum.diode.diodeReverseIV.constant  diode_IfMat=[.07, .12, .19, 1.75, 4.24, 7.32, 11.2; .16, .3, .72, 2.14, 4.02, 6.35, 9.12] % Parameter not set A  diode_VfMat=[0 3.93919 4.34166 5.03764 5.72176 6.19029 7.12243 7.9435 8.58508 9.13853 9.62104 10.0233;0 3.40354 3.71573 4.29235 4.91641 5.38167 6.38957 7.34226 8.07348 8.65657 9.13334 9.54153;0 2.99679 3.29251 3.84591 4.43945 4.88555 5.86847 6.80976 7.53945 8.14153 8.65715 9.11245;0 2.39743 2.63401 3.07672 3.55156 3.90844 4.69478 5.44781 6.03156 6.51323 6.92572 7.28996] % Wolfspeed XML derived V  diode_TjVec=[-55 25 175 900] % Wolfspeed XML derived degC  diode_VfVec=[.5, .7, .9, 1.3, 1.7, 2.1, 2.5] % Parameter not set V  diode_IfVec=[0 1 2 5 10 15 30 50 70 90 110 130] % Wolfspeed XML derived A  diode_IrMat=[1e-06, 2e-06, 5e-06, 1e-05, 2.5e-05, 5e-05, .0001; 2e-06, 5e-06, 1e-05, 4e-05, 8e-05, .0002, .0005] % Parameter not set A  diode_VrMat=[10, 100, 200, 250, 300, 325, 350; 10, 70, 160, 220, 270, 300, 320] % Parameter not set V  diode_VrVec=[10, 20, 40, 50, 70, 80, 100] % Parameter not set V  diode_IrVec=[1e-06, 2e-06, 5e-06, 1e-05, 2e-05, 5e-05, .0001] % Parameter not set A  diode_Vr=-600 % Parameter not set V  diode_Ls=150 % Parameter not set nH  diode_Erec=0.03 % Parameter not set J  diode_rec_loss_model=ee.enum.diode.reverseRecoveryModel.fixed  diode_ErecVal=0 % Parameter not set J  diode_scaleWithIandV=false  diode_ErecMat=[0 0;0 0] % Wolfspeed XML derived J  diodeErecMat3D=zeros(2, 3, 2) J  diode_TjrecVec=[25 35] % Wolfspeed XML derived degC  diode_IfrecVec=[0 10] % Wolfspeed XML derived A  diodeVrecVec=[0, 100] V  diode_IrecVal=10 % Parameter not set A  diode_VrecVal=10 % Wolfspeed XML derived V  diode_tFilter=1 / 1000 / 100 % Parameter not set s  separateThermalPortForDiode=false  thermal_network_parameterization=ee.enum.thermalNetworkTopology.external  Rth=[.03, .2] % Parameter not set K/W  Rth_Cauer=[0.089671 0.30799 0.22252 0.20902] % Wolfspeed XML derived K/W  Rth_Foster=[.08, .14, .22, .16] % Parameter not set K/W  thermal_mass_parameterization=ee.enum.thermalNetwork.thermalmass  thermal_mass=[3, 25] % Parameter not set J/K  thermal_mass_Cauer=[0.00092793 0.0041354 0.020593 0.15749] % Wolfspeed XML derived J/K  thermal_mass_Foster=[.001, .005, .05, .5] % Parameter not set J/K  thermal_time_constant=[.1, 5] % Parameter not set s  thermal_time_constant_Cauer=[.1, 1, 5] % Parameter not set s  thermal_time_constant_Foster=[7e-05, .0007, .01, .08] % Parameter not set s  thermal_mass_initial_temperatures=[25, 25] % Parameter not set degC  thermal_mass_initial_temperatures_Cauer=[25 25 25 25] % Wolfspeed XML derived degC  junction_thermal_mass=0.1 % Parameter not set J/K  Tvec_initial_Foster=[25, 25, 25, 25] % Parameter not set degC  RthDiode=[.03, .2] % Parameter not set K/W  RthCauerDiode=[0.089671 0.30799 0.22252 0.20902] % Wolfspeed XML derived K/W  RthFosterDiode=[.03, .2] % Parameter not set K/W  thermalMassDiode=[3, 25] % Parameter not set J/K  thermalMassCauerDiode=[0.00092793 0.0041354 0.020593 0.15749] % Wolfspeed XML derived J/K  thermalMassFosterDiode=[33, 50] % Parameter not set J/K  thermalTauDiode=[.1, 5] % Parameter not set s  thermalTauCauerDiode=[.1, 1, 5] % Parameter not set s  thermalTauFosterDiode=[1, 10] % Parameter not set s  thermalMassInitTempDiode=[25, 25] % Parameter not set degC  thermalMassInitTempCauerDiode=[25 25 25 25] % Wolfspeed XML derived degC  junctionthermalMassDiode=0.1 % Parameter not set J/K  TVecInitialFosterDiode=[25, 25, 25, 25] % Parameter not set degC  no_thermal_network=0 % Parameter not set  mosfet_junction_temperature_specify=on  mosfet_junction_temperature_priority=High  mosfet_junction_temperature=simTempSec_K K  mosfet_junction_temperature_nominal_specify=off  mosfet_junction_temperature_nominal_value=1  mosfet_junction_temperature_nominal_unit=degC  diode_junction_temperature_specify=off  diode_junction_temperature_priority=None  diode_junction_temperature=simTempSec_K K  diode_junction_temperature_nominal_specify=off  diode_junction_temperature_nominal_value=1  diode_junction_temperature_nominal_unit=degC  Qj_specify=off  Qj_priority=None  Qj=0 W  Qj_nominal_specify=off  Qj_nominal_value=1  Qj_nominal_unit=W  accumulatedSwitchingLosses_specify=off  accumulatedSwitchingLosses_priority=None  accumulatedSwitchingLosses=0 J
  SL_PS{1..4} (4 alike) : nesl_utility/Simulink-PS Converter  PhysicalDomain=network_engine_domain  SubClassName=ps_input  LeftPortType=input  RightPortType=output  PseudoPeriodic=off  Frequencies=[]  NoiseDistribution=none  NoiseParameters=[]  Unit=1  AffineConversion=off  FilteringAndDerivatives=provide  SimscapeFilterOrder=1  InputFilterTimeConstant=0.001  UdotUserProvided=0
  Temperature Source : fl_lib/Thermal/Thermal Sources/Temperature Source  temperature=simTempSec_K K
  Thermal Resistor{1..4} (4 alike) : ee_lib/Passive/Thermal/Thermal Resistor  R=1e-3 K/W  T_specify=on  T_priority=None  T=0 K  T_nominal_specify=off  T_nominal_value=1  T_nominal_unit=K  Q_specify=off  Q_priority=None  Q=0 W  Q_nominal_specify=off  Q_nominal_value=1  Q_nominal_unit=W
  VoutP : PMIOPort  Side=Left
  VoutN : PMIOPort  Port=2  Side=Left
  MidC : PMIOPort  Port=3  Side=Right
  MidD : PMIOPort  Port=4  Side=Right
  wires:
  [G4] -> SL_PS4/1
  [G3] -> SL_PS3/1
  [G2] -> SL_PS2/1
  [G1] -> SL_PS1/1
  Demux/4 -> [G4]
  Demux/3 -> [G3]
  Demux/2 -> [G2]
  Demux/1 -> [G1]
  G/1 -> Demux/1
  connections:
  MOSFETSecA2/RConn2 -- Cds2/RConn1 -- VoutN/RConn1 -- Cds4/RConn1 -- MOSFETSecB2/RConn2
  Thermal Resistor3/LConn1 -- Thermal Resistor1/LConn1 -- Temperature Source/LConn1 -- Thermal Resistor2/LConn1 -- Thermal Resistor4/LConn1
  Thermal Resistor1/RConn1 -- MOSFETSecA2/LConn2
  Thermal Resistor4/RConn1 -- MOSFETSecB2/LConn2
  MOSFETSecA2/RConn1 -- Cds2/LConn1 -- MidC/RConn1 -- Cds1/RConn1 -- MOSFETSecA1/RConn2
  MOSFETSecB2/RConn1 -- Cds4/LConn1 -- MidD/RConn1 -- Cds3/RConn1 -- MOSFETSecB1/RConn2
  Thermal Resistor2/RConn1 -- MOSFETSecA1/LConn2
  MOSFETSecA1/RConn1 -- Cds1/LConn1 -- MOSFETSecB1/RConn1 -- Cds3/LConn1 -- VoutP/RConn1
  SL_PS1/RConn1 -- MOSFETSecA1/LConn1
  SL_PS2/RConn1 -- MOSFETSecA2/LConn1
  SL_PS3/RConn1 -- MOSFETSecB1/LConn1
  SL_PS4/RConn1 -- MOSFETSecB2/LConn1
  MOSFETSecB1/LConn2 -- Thermal Resistor3/RConn1

== system ConverterPlantLibrary/Soft-Switching Converters/DAB Converter/DABConverterVariant/SimplifiedModel/Lr/ExternalInductance ==
  Lr : fl_lib/Electrical/Electrical Elements/Inductor  l=Lr_SI H  r=RLr_SI Ohm  g=1e-05 1/Ohm  i_specify=off  i_priority=None  i=0 A  i_nominal_specify=off  i_nominal_value=1  i_nominal_unit=A  v_specify=off  v_priority=None  v=0 V  v_nominal_specify=off  v_nominal_value=1  v_nominal_unit=V  i_L_specify=off  i_L_priority=High  i_L=0 A  i_L_nominal_specify=off  i_L_nominal_value=1  i_L_nominal_unit=A
  P : PMIOPort  Side=Left
  N : PMIOPort  Port=2  Side=Right
  connections:
  P/RConn1 -- Lr/LConn1
  Lr/RConn1 -- N/RConn1

== system ConverterPlantLibrary/Soft-Switching Converters/DAB Converter/DABConverterVariant/SimplifiedModel/Lr/LeakageInductance ==
  P : PMIOPort  Side=Left
  N : PMIOPort  Port=2  Side=Right
  connections:
  P/RConn1 -- N/RConn1

== system ConverterPlantLibrary/Soft-Switching Converters/LLC Converter/LLC Primary Inverter and Resonant Tank/LLC Detailed Model/Inverter/Iin ==
  Current Sensor : fl_lib/Electrical/Electrical Sensors/Current Sensor
  PS-Simulink Converter : nesl_utility/PS-Simulink Converter  PhysicalDomain=network_engine_domain  SubClassName=ps_output  LeftPortType=input  RightPortType=output  PseudoPeriodic=off  Frequencies=[]  VectorFormat=inherit  Unit=inherit  AffineConversion=off
  + : PMIOPort  Side=Left
  - : PMIOPort  Port=2  Side=Right
  I : Outport
  wires:
  PS-Simulink Converter/1 -> I/1
  connections:
  Current Sensor/RConn1 -- PS-Simulink Converter/LConn1
  +/RConn1 -- Current Sensor/LConn1
  Current Sensor/RConn2 -- -/RConn1

== system ConverterPlantLibrary/Soft-Switching Converters/LLC Converter/LLC Primary Inverter and Resonant Tank/LLC Detailed Model/Inverter/Primary Inverter ==
  G1 : Inport
  G2 : Inport  Port=2
  G3 : Inport  Port=3
  G4 : Inport  Port=4
  Full Bridge with Thermal : Subsystem  VariantControl=FullBridgewithThermal
      settings: PortSchema="{\"entries\":[{\"content\":{\"sides\":[{\"content\":{\"connectorIds\":[\"LConn1\",\"LConn2\"]},\"type\":\"ConnectorPlacement.EquallySpacedRectSide\",\"uuid\":\"27c41940-d662-4779-afdd-48b642f77411\"},{\"content\":{\"connectorIds\":[\"RConn1\",\"RConn2\"],\"side\":\"RIGHT\"},\"type\":\"ConnectorPlacement.EquallySpacedRectSide\",\"uuid\":\"b0072b01-add1-4b0f-b94e-e1b6c9886b0e\"},{\"content\":{\"connectorIds\":[\"In1\",\"In2\",\"In3\",\"In4\"],\"side\":\"TOP\"},\"type\":\"ConnectorPlacement.EquallySpacedRectSide\",\"uuid\":\"c43bed80-422d-49db-9596-8b38d5c3e411\"},{\"content\":{\"side\":\"BOTTOM\"},\"type\":\"ConnectorPlacement.EquallySpacedRectSide\",\"uuid\":\"01f06046-f57e-45b0-bca5-368a5a543f97\"}]},\"type\":\"ConnectorPlacement.EquallySpacedConnector\",\"uuid\":\"2fcb5370-6bd7-4702-bf87-ebedbb7e376c\"}],\"packageUris\":[\"http://schema.mathworks.com/mf0/Connector/R2020b\"],\"version\":\"1.0\"}"
  Half Bridge with Thermal : Subsystem  VariantControl=HalfBridgewithThermal
      settings: PortSchema="{\"entries\":[{\"content\":{\"sides\":[{\"content\":{\"connectorIds\":[\"LConn1\",\"LConn2\"]},\"type\":\"ConnectorPlacement.EquallySpacedRectSide\",\"uuid\":\"27c41940-d662-4779-afdd-48b642f77411\"},{\"content\":{\"connectorIds\":[\"RConn1\",\"RConn2\"],\"side\":\"RIGHT\"},\"type\":\"ConnectorPlacement.EquallySpacedRectSide\",\"uuid\":\"b0072b01-add1-4b0f-b94e-e1b6c9886b0e\"},{\"content\":{\"connectorIds\":[\"In1\",\"In2\",\"In3\",\"In4\"],\"side\":\"TOP\"},\"type\":\"ConnectorPlacement.EquallySpacedRectSide\",\"uuid\":\"c43bed80-422d-49db-9596-8b38d5c3e411\"},{\"content\":{\"side\":\"BOTTOM\"},\"type\":\"ConnectorPlacement.EquallySpacedRectSide\",\"uuid\":\"01f06046-f57e-45b0-bca5-368a5a543f97\"}]},\"type\":\"ConnectorPlacement.EquallySpacedConnector\",\"uuid\":\"2fcb5370-6bd7-4702-bf87-ebedbb7e376c\"}],\"packageUris\":[\"http://schema.mathworks.com/mf0/Connector/R2020b\"],\"version\":\"1.0\"}"
  Ideal Switch Full Bridge : Subsystem  VariantControl=FullBridgewithoutThermal
      settings: PortSchema="{\"entries\":[{\"content\":{\"sides\":[{\"content\":{\"connectorIds\":[\"LConn1\",\"LConn2\"]},\"type\":\"ConnectorPlacement.EquallySpacedRectSide\",\"uuid\":\"27c41940-d662-4779-afdd-48b642f77411\"},{\"content\":{\"connectorIds\":[\"RConn1\",\"RConn2\"],\"side\":\"RIGHT\"},\"type\":\"ConnectorPlacement.EquallySpacedRectSide\",\"uuid\":\"b0072b01-add1-4b0f-b94e-e1b6c9886b0e\"},{\"content\":{\"connectorIds\":[\"In1\",\"In2\",\"In3\",\"In4\"],\"side\":\"TOP\"},\"type\":\"ConnectorPlacement.EquallySpacedRectSide\",\"uuid\":\"c43bed80-422d-49db-9596-8b38d5c3e411\"},{\"content\":{\"side\":\"BOTTOM\"},\"type\":\"ConnectorPlacement.EquallySpacedRectSide\",\"uuid\":\"01f06046-f57e-45b0-bca5-368a5a543f97\"}]},\"type\":\"ConnectorPlacement.EquallySpacedConnector\",\"uuid\":\"2fcb5370-6bd7-4702-bf87-ebedbb7e376c\"}],\"packageUris\":[\"http://schema.mathworks.com/mf0/Connector/R2020b\"],\"version\":\"1.0\"}"
  Ideal Switch Half Bridge : Subsystem  VariantControl=HalfBridgewithoutThermal
      settings: PortSchema="{\"entries\":[{\"content\":{\"sides\":[{\"content\":{\"connectorIds\":[\"LConn1\",\"LConn2\"]},\"type\":\"ConnectorPlacement.EquallySpacedRectSide\",\"uuid\":\"27c41940-d662-4779-afdd-48b642f77411\"},{\"content\":{\"connectorIds\":[\"RConn1\",\"RConn2\"],\"side\":\"RIGHT\"},\"type\":\"ConnectorPlacement.EquallySpacedRectSide\",\"uuid\":\"b0072b01-add1-4b0f-b94e-e1b6c9886b0e\"},{\"content\":{\"connectorIds\":[\"In1\",\"In2\",\"In3\",\"In4\"],\"side\":\"TOP\"},\"type\":\"ConnectorPlacement.EquallySpacedRectSide\",\"uuid\":\"c43bed80-422d-49db-9596-8b38d5c3e411\"},{\"content\":{\"side\":\"BOTTOM\"},\"type\":\"ConnectorPlacement.EquallySpacedRectSide\",\"uuid\":\"01f06046-f57e-45b0-bca5-368a5a543f97\"}]},\"type\":\"ConnectorPlacement.EquallySpacedConnector\",\"uuid\":\"2fcb5370-6bd7-4702-bf87-ebedbb7e376c\"}],\"packageUris\":[\"http://schema.mathworks.com/mf0/Connector/R2020b\"],\"version\":\"1.0\"}"
  P1 : PMIOPort  Side=Left
  N1 : PMIOPort  Port=2  Side=Left
  P2 : PMIOPort  Port=3  Side=Right
  N2 : PMIOPort  Port=4  Side=Right

== system ConverterPlantLibrary/Soft-Switching Converters/LLC Converter/LLC Primary Inverter and Resonant Tank/LLC Detailed Model/Inverter/Vin ==
  PS-Simulink Converter : nesl_utility/PS-Simulink Converter  PhysicalDomain=network_engine_domain  SubClassName=ps_output  LeftPortType=input  RightPortType=output  PseudoPeriodic=off  Frequencies=[]  VectorFormat=inherit  Unit=inherit  AffineConversion=off
  Voltage Sensor : fl_lib/Electrical/Electrical Sensors/Voltage Sensor
  + : PMIOPort  Side=Left
  - : PMIOPort  Port=2  Side=Right
  V : Outport
  wires:
  PS-Simulink Converter/1 -> V/1
  connections:
  PS-Simulink Converter/LConn1 -- Voltage Sensor/RConn1
  Voltage Sensor/LConn1 -- +/RConn1
  Voltage Sensor/RConn2 -- -/RConn1

== system ConverterPlantLibrary/Soft-Switching Converters/LLC Converter/LLC Primary Inverter and Resonant Tank/LLC Detailed Model/Resonant Tank/Ip ==
  Current Sensor : fl_lib/Electrical/Electrical Sensors/Current Sensor
  PS-Simulink Converter : nesl_utility/PS-Simulink Converter  PhysicalDomain=network_engine_domain  SubClassName=ps_output  LeftPortType=input  RightPortType=output  PseudoPeriodic=off  Frequencies=[]  VectorFormat=inherit  Unit=inherit  AffineConversion=off
  + : PMIOPort  Side=Left
  - : PMIOPort  Port=2  Side=Right
  I : Outport
  wires:
  PS-Simulink Converter/1 -> I/1
  connections:
  Current Sensor/RConn1 -- PS-Simulink Converter/LConn1
  +/RConn1 -- Current Sensor/LConn1
  Current Sensor/RConn2 -- -/RConn1

== system ConverterPlantLibrary/Soft-Switching Converters/LLC Converter/LLC Primary Inverter and Resonant Tank/LLC Detailed Model/Resonant Tank/Lr ==
  ExternalInductance : Subsystem  VariantControl=ExternalInductance
  LeakageInductance : Subsystem  VariantControl=LeakageInductance
  P : PMIOPort  Side=Left
  N : PMIOPort  Port=2  Side=Right

== system ConverterPlantLibrary/Soft-Switching Converters/LLC Converter/LLC Primary Inverter and Resonant Tank/LLC Detailed Model/Resonant Tank/Vp ==
  PS-Simulink Converter : nesl_utility/PS-Simulink Converter  PhysicalDomain=network_engine_domain  SubClassName=ps_output  LeftPortType=input  RightPortType=output  PseudoPeriodic=off  Frequencies=[]  VectorFormat=inherit  Unit=inherit  AffineConversion=off
  Voltage Sensor : fl_lib/Electrical/Electrical Sensors/Voltage Sensor
  + : PMIOPort  Side=Left
  - : PMIOPort  Port=2  Side=Right
  V : Outport
  wires:
  PS-Simulink Converter/1 -> V/1
  connections:
  PS-Simulink Converter/LConn1 -- Voltage Sensor/RConn1
  Voltage Sensor/LConn1 -- +/RConn1
  Voltage Sensor/RConn2 -- -/RConn1

== system ConverterPlantLibrary/Soft-Switching Converters/LLC Converter/LLC Primary Inverter and Resonant Tank/LLC Detailed Model/Resonant Tank/Vs ==
  PS-Simulink Converter : nesl_utility/PS-Simulink Converter  PhysicalDomain=network_engine_domain  SubClassName=ps_output  LeftPortType=input  RightPortType=output  PseudoPeriodic=off  Frequencies=[]  VectorFormat=inherit  Unit=inherit  AffineConversion=off
  Voltage Sensor : fl_lib/Electrical/Electrical Sensors/Voltage Sensor
  + : PMIOPort  Side=Left
  - : PMIOPort  Port=2  Side=Right
  V : Outport
  wires:
  PS-Simulink Converter/1 -> V/1
  connections:
  PS-Simulink Converter/LConn1 -- Voltage Sensor/RConn1
  Voltage Sensor/LConn1 -- +/RConn1
  Voltage Sensor/RConn2 -- -/RConn1
